simulink model "pid_init_nonleaner"  (R2024b)
settings: Solver=VariableStepAuto  StartTime=0.0  StopTime=3.14  RelTol=1e-3
libraries: slpidlib x2, simulink x2
settings Model: Creator=rezax  LastModifiedBy=rezax

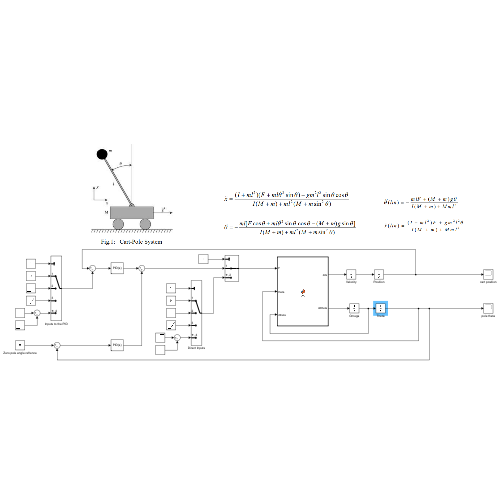
[thumbnail: Simulink's stored preview of the top-level diagram]
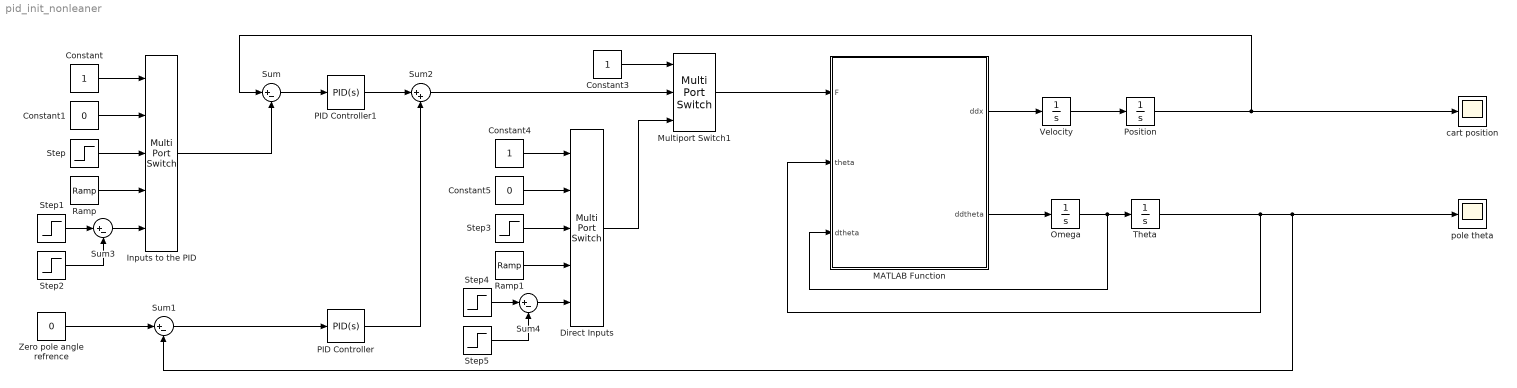
== system pid_init_nonleaner ==
  Constant : Constant
  Constant1 : Constant  Value=0
  Constant3 : Constant
  Constant4 : Constant
  Constant5 : Constant  Value=0
  Direct Inputs : MultiPortSwitch  Inputs=4  SaturateOnIntegerOverflow=off  InputSameDT=off
  Inputs to the PID : MultiPortSwitch  Inputs=4  SaturateOnIntegerOverflow=off  InputSameDT=off
  MATLAB Function : MATLAB Function  TreatAsAtomicUnit=on
  Multiport Switch1 : MultiPortSwitch  Inputs=2  SaturateOnIntegerOverflow=off  InputSameDT=off
  Omega : Integrator
  PID Controller : slpidlib/PID Controller  Controller=PID  Form=Parallel  TimeDomain=Continuous-time  UseExternalTs=off  SampleTime=-1  IntegratorMethod=Forward Euler  FilterMethod=Forward Euler  ControllerParametersSource=internal  P=-500  I=-1  UseKiTs=off  D=-100  UseExternalDerivativeSource=off  N=100  UseFilter=on  TunerSelectOption=Frequency Response Based  InitialConditionSource=internal  InitialConditionForIntegrator=0  InitialConditionForFilter=0  DifferentiatorICPrevScaledInput=0  ExternalReset=none  TrackingMode=off  Kt=1  LimitOutput=off  SatLimitsSource=internal  UpperSaturationLimit=inf  LowerSaturationLimit=-inf  LinearizeAsGain=on  AntiWindupMode=none  Kb=1  LimitIntegrator=off  UpperIntegratorSaturationLimit=inf  LowerIntegratorSaturationLimit=-inf  POutMin=[]  POutMax=[]  IOutMin=[]  IOutMax=[]  DOutMin=[]  DOutMax=[]  NOutMin=[]  NOutMax=[]  SumOutMin=[]  SumOutMax=[]  SaturationOutMin=[]  SaturationOutMax=[]  PParamMin=[]  PParamMax=[]  IParamMin=[]  IParamMax=[]  DParamMin=[]  DParamMax=[]  NParamMin=[]  NParamMax=[]  KbParamMin=[]  KbParamMax=[]  KtParamMin=[]  KtParamMax=[]  KbOutMin=[]  KbOutMax=[]  KtOutMin=[]  KtOutMax=[]  IntegratorOutMin=[]  IntegratorOutMax=[]  FilterOutMin=[]  FilterOutMax=[]  SumI1OutMin=[]  SumI1OutMax=[]  SumI2OutMin=[]  SumI2OutMax=[]  SumI3OutMin=[]  SumI3OutMax=[]  SumI4OutMin=[]  SumI4OutMax=[]  SumDOutMin=[]  SumDOutMax=[]  DifferentiatorOutMin=[]  DifferentiatorOutMax=[]  FilterDiffOutCoefMin=[]  FilterDiffOutCoefMax=[]  ReciprocalOutMin=[]  ReciprocalOutMax=[]  SumDenOutMin=[]  SumDenOutMax=[]  SumNumOutMin=[]  SumNumOutMax=[]  DivideOutMin=[]  DivideOutMax=[]  UdiffTsProdOutMin=[]  UdiffTsProdOutMax=[]  NTsProdOutMin=[]  NTsProdOutMax=[]  UintegralTsProdOutMin=[]  UintegralTsProdOutMax=[]  UngainTsProdOutMin=[]  UngainTsProdOutMax=[]  ClampingZeroOutDataTypeStr=Inherit: Inherit via back propagation  ClampingZeroOutMin=[]  ClampingZeroOutMax=[]  FilterDenConstantOutDataTypeStr=Inherit: Inherit via back propagation  FilterDenConstantOutMin=[]  FilterDenConstantOutMax=[]  PCopyOutDataTypeStr=Inherit: Inherit via back propagation  PCopyOutMin=[]  PCopyOutMax=[]  NCopyOutDataTypeStr=Inherit: Inherit via back propagation  NCopyOutMin=[]  NCopyOutMax=[]  IntegratorContinuousStateAttributes=''  IntegratorStateMustResolveToSignalObject=off  IntegratorRTWStateStorageClass=Auto  FilterContinuousStateAttributes=''  FilterStateMustResolveToSignalObject=off  FilterRTWStateStorageClass=Auto  ParallelPVariant=InternalParameters  IdealPVariant=Disabled  IVariant=InternalParameters  DVariant=InternalParameters  IntegratorVariant=Continuous  SatVariant=Disabled  AWVariant=Passthrough  PCopyVariant=Disabled  TRVariant=Disabled  FdbkBlocksVariant=Forward  IdealPFdbkVariant=Disabled  SatFdbkVariant=Disabled  DerivativeFilterVariant=ContFilter  NVariant=InternalParameters  NCopyVariant=Disabled  FilterICVariant=InternalICsFilter  IntegratorICVariant=InternalICs  ExternalResetVariant=Disabled  TRSumVariant=Passthrough  SumFdbkVariant=Disabled  SumVariant=Sum_PID  TsampFilterVariant=InternalTs  TsampNgainVariant=Passthrough  TsampIntegralVariant=Disabled_SignalSpec  ExternalSaturationOutDataTypeStr=Inherit: Same as second input  DerivativeSourceVariant=ErrorSignal  PreIntVariant=InternalPreInt
  PID Controller1 : slpidlib/PID Controller  Controller=PID  Form=Parallel  TimeDomain=Continuous-time  UseExternalTs=off  SampleTime=-1  IntegratorMethod=Forward Euler  FilterMethod=Forward Euler  ControllerParametersSource=internal  P=40  I=0.8  UseKiTs=off  D=28  UseExternalDerivativeSource=off  N=100  UseFilter=on  TunerSelectOption=Transfer Function Based (PID Tuner App)  InitialConditionSource=internal  InitialConditionForIntegrator=0  InitialConditionForFilter=0  DifferentiatorICPrevScaledInput=0  ExternalReset=none  TrackingMode=off  Kt=1  LimitOutput=off  SatLimitsSource=internal  UpperSaturationLimit=inf  LowerSaturationLimit=-inf  LinearizeAsGain=on  AntiWindupMode=none  Kb=1  LimitIntegrator=off  UpperIntegratorSaturationLimit=inf  LowerIntegratorSaturationLimit=-inf  POutMin=[]  POutMax=[]  IOutMin=[]  IOutMax=[]  DOutMin=[]  DOutMax=[]  NOutMin=[]  NOutMax=[]  SumOutMin=[]  SumOutMax=[]  SaturationOutMin=[]  SaturationOutMax=[]  PParamMin=[]  PParamMax=[]  IParamMin=[]  IParamMax=[]  DParamMin=[]  DParamMax=[]  NParamMin=[]  NParamMax=[]  KbParamMin=[]  KbParamMax=[]  KtParamMin=[]  KtParamMax=[]  KbOutMin=[]  KbOutMax=[]  KtOutMin=[]  KtOutMax=[]  IntegratorOutMin=[]  IntegratorOutMax=[]  FilterOutMin=[]  FilterOutMax=[]  SumI1OutMin=[]  SumI1OutMax=[]  SumI2OutMin=[]  SumI2OutMax=[]  SumI3OutMin=[]  SumI3OutMax=[]  SumI4OutMin=[]  SumI4OutMax=[]  SumDOutMin=[]  SumDOutMax=[]  DifferentiatorOutMin=[]  DifferentiatorOutMax=[]  FilterDiffOutCoefMin=[]  FilterDiffOutCoefMax=[]  ReciprocalOutMin=[]  ReciprocalOutMax=[]  SumDenOutMin=[]  SumDenOutMax=[]  SumNumOutMin=[]  SumNumOutMax=[]  DivideOutMin=[]  DivideOutMax=[]  UdiffTsProdOutMin=[]  UdiffTsProdOutMax=[]  NTsProdOutMin=[]  NTsProdOutMax=[]  UintegralTsProdOutMin=[]  UintegralTsProdOutMax=[]  UngainTsProdOutMin=[]  UngainTsProdOutMax=[]  ClampingZeroOutDataTypeStr=Inherit: Inherit via back propagation  ClampingZeroOutMin=[]  ClampingZeroOutMax=[]  FilterDenConstantOutDataTypeStr=Inherit: Inherit via back propagation  FilterDenConstantOutMin=[]  FilterDenConstantOutMax=[]  PCopyOutDataTypeStr=Inherit: Inherit via back propagation  PCopyOutMin=[]  PCopyOutMax=[]  NCopyOutDataTypeStr=Inherit: Inherit via back propagation  NCopyOutMin=[]  NCopyOutMax=[]  IntegratorContinuousStateAttributes=''  IntegratorStateMustResolveToSignalObject=off  IntegratorRTWStateStorageClass=Auto  FilterContinuousStateAttributes=''  FilterStateMustResolveToSignalObject=off  FilterRTWStateStorageClass=Auto  ParallelPVariant=InternalParameters  IdealPVariant=Disabled  IVariant=InternalParameters  DVariant=InternalParameters  IntegratorVariant=Continuous  SatVariant=Disabled  AWVariant=Passthrough  PCopyVariant=Disabled  TRVariant=Disabled  FdbkBlocksVariant=Forward  IdealPFdbkVariant=Disabled  SatFdbkVariant=Disabled  DerivativeFilterVariant=ContFilter  NVariant=InternalParameters  NCopyVariant=Disabled  FilterICVariant=InternalICsFilter  IntegratorICVariant=InternalICs  ExternalResetVariant=Disabled  TRSumVariant=Passthrough  SumFdbkVariant=Disabled  SumVariant=Sum_PID  TsampFilterVariant=InternalTs  TsampNgainVariant=Passthrough  TsampIntegralVariant=Disabled_SignalSpec  ExternalSaturationOutDataTypeStr=Inherit: Same as second input  DerivativeSourceVariant=ErrorSignal  PreIntVariant=InternalPreInt
  Position : Integrator
  Ramp : simulink/Sources/Ramp  slope=1  start=0  InitialOutput=0
  Ramp1 : simulink/Sources/Ramp  slope=1  start=0  InitialOutput=0
  Step : Step  Time=0  SampleTime=0
  Step1 : Step  SampleTime=0
  Step2 : Step  Time=1.05  SampleTime=0
  Step3 : Step  Time=0  SampleTime=0
  Step4 : Step  SampleTime=0
  Step5 : Step  Time=1.05  SampleTime=0
  Sum{,1,3..4} (4 alike) : Sum  Inputs=|+-
  Sum2 : Sum  Inputs=|++
  Theta : Integrator  InitialCondition=0.05
  Velocity : Integrator
  Zero pole angle refrence : Constant  Value=0
  cart position : Scope
  pole theta : Scope
  wires:
  MATLAB Function/2(ddtheta) -> Omega/1
  Omega/1 -> MATLAB Function/3(dtheta), Theta/1
  MATLAB Function/1(ddx) -> Velocity/1
  Velocity/1 -> Position/1
  Theta/1 -> MATLAB Function/2(theta), pole theta/1, Sum1/2
  Position/1 -> Sum/1, cart position/1
  Sum1/1 -> PID Controller/1
  PID Controller/1 -> Sum2/2
  Sum/1 -> PID Controller1/1
  Sum2/1 -> Multiport Switch1/2
  Constant/1 -> Inputs to the PID/1
  Constant1/1 -> Inputs to the PID/2
  Step/1 -> Inputs to the PID/3
  Ramp/1 -> Inputs to the PID/4
  Step1/1 -> Sum3/1
  Step2/1 -> Sum3/2
  Sum3/1 -> Inputs to the PID/5
  Inputs to the PID/1 -> Sum/2
  Zero pole angle refrence/1 -> Sum1/1
  Constant3/1 -> Multiport Switch1/1
  Multiport Switch1/1 -> MATLAB Function/1(F)
  Ramp1/1 -> Direct Inputs/4
  Step3/1 -> Direct Inputs/3
  Constant4/1 -> Direct Inputs/1
  Constant5/1 -> Direct Inputs/2
  Step4/1 -> Sum4/1
  Sum4/1 -> Direct Inputs/5
  Step5/1 -> Sum4/2
  Direct Inputs/1 -> Multiport Switch1/3
  PID Controller1/1 -> Sum2/1

== matlab function pid_init_nonleaner/MATLAB Function ==
  data: F input; ddx output; theta input; dtheta input; ddtheta output
function [ddx, ddtheta] = fcn(F, theta, dtheta)
% Non-Linear Cart-Pole Dynamics
% Inputs: F (Force), theta (Angle), dtheta (Angular Velocity)

% Parameters
M = 2.0; m = 0.2; l = 0.5; g = 9.81; I = 0.099;

% Trig functions
s = sin(theta);
c = cos(theta);

% Common Denominator
D = (M + m)*(I + m*l^2) - (m*l*c)^2;

% Cart Acceleration (ddx)
num_x = (I + m*l^2)*(F + m*l*dtheta^2*s) - (m*l*c)*(m*g*l*s);
ddx = num_x / D;

% Angular Acceleration (ddtheta)
num_theta = (M + m)*(m*g*l*s) - (m*l*c)*(F + m*l*dtheta^2*s);
ddtheta = num_theta / D;
